simulink model "afe_dqctrl_param"  (R2026a)
settings: Solver=ode23tb  StopTime=param.sim.simlength  FixedStep=tc  MaxStep=param.glb_time.tc
values from neighbouring files (symbols this model uses):
  param = add_template_extras(param, options)    [init_model.m]
undefined symbols (not defined in the file or in its folder): magnitude
libraries: fl_lib x166, nesl_utility x91, igbt_simple_2th_lib x6, single_phase_transformer_lib x3, discrete_time_low_pass_filter x1, threephase_inductor_lib x1, dclink_for_two_levels x1, three_phase_pwm_modulator x1, three_phase_voltage_with_frt_emulator x1
(part 3 of 7)

== system afe_dqctrl_param/afe_dq_mod1/AFE_control/afe_control/acquisitions/ug afe quantizzation and one step delay ==
  ug_abc_pu : Inport
  Demux : Demux  Outputs=3
  Mux : Mux  Inputs=3
  ug afe quantizzation and one step delay : Subsystem
  ugd_abc_pu : Outport
  wires:
  ug afe quantizzation and one step delay/2(ugd_v_pu) -> Mux/2
  Demux/2 -> ug afe quantizzation and one step delay/2(ug_v_pu)
  Demux/3 -> ug afe quantizzation and one step delay/3(ug_w_pu)
  ug afe quantizzation and one step delay/1(ugd_u_pu) -> Mux/1
  Demux/1 -> ug afe quantizzation and one step delay/1(ug_u_pu)
  ug_abc_pu/1 -> Demux/1
  ug afe quantizzation and one step delay/3(ugd_w_pu) -> Mux/3
  Mux/1 -> ugd_abc_pu/1

== system afe_dqctrl_param/afe_dq_mod1/AFE_control/afe_control/current_ctrl/current_transformation ==
  is_a_pu : Inport
  is_b_pu : Inport  Port=2
  is_c_pu : Inport  Port=3
  alphabeta2xieta : MATLAB Function  TreatAsAtomicUnit=on
  uvw2alphabeta : MATLAB Function  TreatAsAtomicUnit=on
  tag scope: id_eta_pu=scoped, id_xi_pu=scoped
  wires:
  is_c_pu/1 -> uvw2alphabeta/3(w)
  alphabeta2xieta/2(eta) -> [id_eta_pu]  "ieta_pu"
  alphabeta2xieta/1(xi) -> [id_xi_pu]  "ixi_pu"
  is_b_pu/1 -> uvw2alphabeta/2(v)
  uvw2alphabeta/2(beta) -> alphabeta2xieta/2(beta)  "ibeta_pu"
  uvw2alphabeta/1(alpha) -> alphabeta2xieta/1(alpha)  "ialpha_pu"
  [phase_grid_pll] -> alphabeta2xieta/3(gamma)
  is_a_pu/1 -> uvw2alphabeta/1(u)

== system afe_dqctrl_param/afe_dq_mod1/AFE_control/afe_control/current_ctrl/dq_vector_pi ==
  id : Inport
  id_ref : Inport  Port=2
  iq : Inport  Port=3
  iq_ref : Inport  Port=4
  Sum1 : Sum  Inputs=|-+
  Sum2 : Sum  Inputs=|-+
  bounder1 : Subsystem
  bounder2 : Subsystem
  pi_d : Subsystem
  pi_q : Subsystem
  switch : Subsystem
  vector lenght : Subsystem
  md_sat : Outport
  mq_sat : Outport  Port=2
  wires:
  bounder2/2(clip) -> switch/2(clip 2)
  vector lenght/2(m) -> bounder1/3(m), bounder2/1(m)
  Sum2/1 -> pi_q/1(iq_tilde)
  pi_d/1(ud_out) -> vector lenght/1(md), bounder1/1(md)
  pi_q/1(Vqs_out) -> bounder2/3(mq), vector lenght/2(mq)
  vector lenght/1(m_1) -> bounder1/2(m_1), bounder2/2(m_1)
  switch/1(clip) -> pi_q/2(clip), pi_d/2(clip)
  iq/1 -> Sum2/1
  Sum1/1 -> pi_d/1(id_tilde)
  bounder1/2(clip) -> switch/1(clip 1)
  id/1 -> Sum1/1
  bounder1/1(md_sat) -> md_sat/1
  bounder2/1(mq_sat) -> mq_sat/1
  id_ref/1 -> Sum1/2
  iq_ref/1 -> Sum2/2

== system afe_dqctrl_param/afe_dq_mod1/AFE_control/afe_control/current_ctrl/zero_current_ctrl ==
  ualpha_ctrl_afe : Inport
  ubeta_ctrl_afe : Inport  Port=2
  Bus Creator1 : BusCreator  Inputs=3
  iz : Subsystem
  zero_sequence_current_ctrl : Subsystem
  uabg_ctrl_out : Outport
  wires:
  Bus Creator1/1 -> uabg_ctrl_out/1
  ualpha_ctrl_afe/1 -> Bus Creator1/1  "ualpha_ctrl_afe"
  ubeta_ctrl_afe/1 -> Bus Creator1/2  "ubeta_ctrl_afe"
  iz/1(iz) -> zero_sequence_current_ctrl/1(iz)
  zero_sequence_current_ctrl/1(ugamma_afe) -> Bus Creator1/3  "ugamma_ctrl_afe"

== system afe_dqctrl_param/afe_dq_mod1/AFE_control/afe_control/data_to_worspace_module_1/dq_pll ==
  Bus Creator1 : BusCreator  Inputs=8
  dqPLLs : Outport
  wires:
  [phase_grid_fht_simulink_pll] -> Bus Creator1/5  "phase_grid_fht_simulink_pll"
  [omega_grid_fht_simulink_pll] -> Bus Creator1/6  "omega_grid_fht_simulink_pll"
  [omega_grid_fhtsr_dqpll] -> Bus Creator1/8  "omega_grid_fhtsr_dqpll"
  [phase_grid_fhtsr_dqpll] -> Bus Creator1/7  "phase_grid_fhtsr_dqpll"
  [omega_grid_dqpll_ccaller] -> Bus Creator1/4  "omega_grid_dqpll_ccaller"
  [phase_grid_dqpll_ccaller] -> Bus Creator1/3  "phase_grid_dqpll_ccaller"
  [omega_grid_pu_dqpll] -> Bus Creator1/2  "omega_grid_pu_dqpll"
  [phase_grid_dqpll] -> Bus Creator1/1  "phase_grid_dqpll"
  Bus Creator1/1 -> dqPLLs/1

== system afe_dqctrl_param/afe_dq_mod1/AFE_control/afe_control/data_to_worspace_module_1/pwr_meter ==
  Bus Creator1 : BusCreator  Inputs=4
  m_pwr_meter : Outport
  wires:
  [u_grid_pu_rms] -> Bus Creator1/2  "u_grid_pu_rms"
  Bus Creator1/1 -> m_pwr_meter/1
  [pwr_act_grid] -> Bus Creator1/3  "pwr_act_grid"
  [pwr_react_grid] -> Bus Creator1/4  "pwr_react_grid"
  [i_grid_pu_rms] -> Bus Creator1/1  "i_grid_pu_rms"

== system afe_dqctrl_param/afe_dq_mod1/AFE_control/afe_control/grid_voltage_phase_lock_loops/FHT-PLL ==
  ug_abc_pu : Inport
  pll_stageA : Subsystem
  pll_stageB : Subsystem
  gamma_grid_fht_pll : Outport
  omega_grid_fht_pll : Outport  Port=2
  wires:
  ug_abc_pu/1 -> pll_stageA/2(ug_abc_pu)
  pll_stageB/2(omega_grid_ddsrf_pll) -> omega_grid_fht_pll/1
  pll_stageA/1(u_grid_xi) -> pll_stageB/1(u_grid_pos_xi)  "u_grid_pos_xi"
  pll_stageA/2(u_grid_eta) -> pll_stageB/2(u_grid_pos_eta)  "u_grid_pos_eta"
  pll_stageB/1(gamma_grid_ddsrf_pll) -> gamma_grid_fht_pll/1, pll_stageA/1(gamma_grid)

== system afe_dqctrl_param/afe_dq_mod1/AFE_control/afe_control/grid_voltage_phase_lock_loops/FHT-PLL_simulink ==
  ug_abc_pu : Inport
  pll_stageA : Subsystem
  pll_stageB : Subsystem
  gamma_grid_fht_pll : Outport
  omega_grid_fht_pll : Outport  Port=2
  wires:
  pll_stageB/1(gamma_grid_ddsrf_pll) -> pll_stageA/1(gamma_grid), gamma_grid_fht_pll/1
  pll_stageA/2(u_grid_eta) -> pll_stageB/2(u_grid_pos_eta)  "u_grid_pos_eta"
  pll_stageA/1(u_grid_xi) -> pll_stageB/1(u_grid_pos_xi)  "u_grid_pos_xi"
  pll_stageB/2(omega_grid_ddsrf_pll) -> omega_grid_fht_pll/1
  ug_abc_pu/1 -> pll_stageA/2(ug_abc_pu)

== system afe_dqctrl_param/afe_dq_mod1/AFE_control/afe_control/grid_voltage_phase_lock_loops/dq_pll ==
  ug_abc_pu : Inport
  Goto Tag Visibility29 : GotoTagVisibility  GotoTag=Vgrid_unorm_dqpll
  pll_stageA : Subsystem
  pll_stageB : Subsystem
  phase_grid_dqpll : Outport
  omega_grid_pu_dqpll : Outport  Port=2
  wires:
  pll_stageA/2(u_grid_pos_eta) -> pll_stageB/2(u_grid_pos_eta)  "u_grid_pos_eta"
  pll_stageB/1(phase_grid_pll) -> phase_grid_dqpll/1, pll_stageA/1(phase_grid)
  pll_stageA/1(u_grid_pos_xi) -> pll_stageB/1(u_grid_pos_xi)  "u_grid_pos_xi"
  pll_stageB/2(omega_grid_pu_pll) -> omega_grid_pu_dqpll/1
  ug_abc_pu/1 -> pll_stageA/2(ug_abc)

== system afe_dqctrl_param/afe_dq_mod1/AFE_control/afe_control/grid_voltage_phase_lock_loops/dq_pll_ccaller ==
  ug_abc_pu : Inport
  Bus Selector : BusSelector  OutputSignals=omega_pu_hat,gamma_hat,u_grid_xi,u_grid_eta,dqpll_pll_state
  C Caller : CCaller  FunctionName=dqpll_grid_process_simulink  PortSpecificationStruct="%)30     .    N H   8    (     @         %    \"     8    !     0         %  0 \"0    $    _    07)G3F%M90  4&]R=$YA;64 4V-O<&4     26YD97@     5'EP90      4VEZ90      27-';&]B86P   X    P    !@    @    $          4    (     0    ,    !         !   P!O=70 #@   #     &    \"     0         !0    @    !     P    $         $  # &]U=  .    .     8    (    !          %    \"     $    &     0         0   ...(+3319 chars)"
  Constant : Constant  Value=param.glb_time.ts_afe
  Data Type Conversion{1..2,4..5} (4 alike) : DataTypeConversion  OutDataTypeStr=single  SaturateOnIntegerOverflow=off  RndMeth=Floor
  Data Type Conversion{6..10} (5 alike) : DataTypeConversion  OutDataTypeStr=double  SaturateOnIntegerOverflow=off  RndMeth=Floor
  Data Type Conversion3 : DataTypeConversion  OutDataTypeStr=uint8  SaturateOnIntegerOverflow=off  RndMeth=Floor
  Demux : Demux  Outputs=3
  Step : Step  Time=0.01  InitialValue=1  FinalValue=0
  first_harmonic_tracker : Scope  NumInputPorts=3
      settings: ActiveDisplayYMinimum=-1.7184470891952515  ActiveDisplayYMaximum=1.8384636640548706
  first_harmonic_tracker_phase_u : Subsystem
  first_harmonic_tracker_phase_v : Subsystem
  first_harmonic_tracker_phase_w : Subsystem
  gamma_hat : Outport  VectorParamsAs1DForOutWhenUnconnected=off
  omega_pu_hat : Outport  Port=2  VectorParamsAs1DForOutWhenUnconnected=off
  dqpll_uxi : Outport  Port=3  VectorParamsAs1DForOutWhenUnconnected=off
  dqpll_ueta : Outport  Port=4  VectorParamsAs1DForOutWhenUnconnected=off
  dqpll_state : Outport  Port=5  VectorParamsAs1DForOutWhenUnconnected=off
  wires:
  Step/1 -> Data Type Conversion3/1
  Constant/1 -> Data Type Conversion1/1
  Data Type Conversion3/1 -> C Caller/1
  Data Type Conversion2/1 -> C Caller/2
  Data Type Conversion4/1 -> C Caller/3
  Data Type Conversion5/1 -> C Caller/4
  Data Type Conversion1/1 -> C Caller/5
  C Caller/1 -> Bus Selector/1
  Bus Selector/1 -> Data Type Conversion6/1  "<omega_pu_hat>"
  Bus Selector/2 -> Data Type Conversion7/1  "<gamma_hat>"
  Bus Selector/3 -> Data Type Conversion8/1  "<u_grid_xi>"
  Bus Selector/4 -> Data Type Conversion9/1  "<u_grid_eta>"
  Bus Selector/5 -> Data Type Conversion10/1  "<dqpll_pll_state>"
  Data Type Conversion7/1 -> gamma_hat/1
  Data Type Conversion10/1 -> dqpll_state/1
  Data Type Conversion8/1 -> dqpll_uxi/1
  Data Type Conversion9/1 -> dqpll_ueta/1
  ug_abc_pu/1 -> Demux/1
  Demux/1 -> first_harmonic_tracker_phase_u/1(u)
  Demux/2 -> first_harmonic_tracker_phase_v/1(u)
  Demux/3 -> first_harmonic_tracker_phase_w/1(u)
  Data Type Conversion6/1 -> omega_pu_hat/1
  first_harmonic_tracker_phase_u/1(u_hat) -> first_harmonic_tracker/1, Data Type Conversion2/1  "tracker_phase_u"
  first_harmonic_tracker_phase_v/1(u_hat) -> first_harmonic_tracker/2, Data Type Conversion4/1  "tracker_phase_v"
  first_harmonic_tracker_phase_w/1(u_hat) -> first_harmonic_tracker/3, Data Type Conversion5/1  "tracker_phase_w"

== system afe_dqctrl_param/afe_dq_mod1/AFE_control/afe_control/instantaneus_power/abc2alphabeta ==
  a : Inport
  b : Inport  Port=2
  c : Inport  Port=3
  Gain1 : Gain  Gain=-1/2
  Gain11 : Gain  Gain=-1/2
  Gain2 : Gain  Gain=0
  Gain3 : Gain  Gain=sqrt(3)/2
  Gain4 : Gain  Gain=-sqrt(3)/2
  Gain8 : Gain  Gain=2/3
  Gain9 : Gain  Gain=2/3
  Sum : Sum  Inputs=+++
  Sum1 : Sum  Inputs=+++
  "alpha " : Outport  VectorParamsAs1DForOutWhenUnconnected=off
  "beta " : Outport  Port=2  VectorParamsAs1DForOutWhenUnconnected=off
  wires:
  Gain3/1 -> Sum1/2
  Gain2/1 -> Sum1/1
  Gain11/1 -> Sum/2
  Gain4/1 -> Sum1/3
  Sum1/1 -> Gain9/1
  Gain8/1 -> "alpha "/1
  Sum/1 -> Gain8/1
  c/1 -> Gain4/1, Gain1/1
  Gain9/1 -> "beta "/1
  b/1 -> Gain3/1, Gain11/1
  Gain1/1 -> Sum/3
  a/1 -> Gain2/1, Sum/1

== system afe_dqctrl_param/afe_dq_mod1/AFE_control/afe_control/instantaneus_power/abc2alphabeta  ==
  a : Inport
  b : Inport  Port=2
  c : Inport  Port=3
  Gain1 : Gain  Gain=-1/2
  Gain11 : Gain  Gain=-1/2
  Gain2 : Gain  Gain=0
  Gain3 : Gain  Gain=sqrt(3)/2
  Gain4 : Gain  Gain=-sqrt(3)/2
  Gain8 : Gain  Gain=2/3
  Gain9 : Gain  Gain=2/3
  Sum : Sum  Inputs=+++
  Sum1 : Sum  Inputs=+++
  "alpha " : Outport  VectorParamsAs1DForOutWhenUnconnected=off
  "beta " : Outport  Port=2  VectorParamsAs1DForOutWhenUnconnected=off
  wires:
  a/1 -> Sum/1, Gain2/1
  Gain2/1 -> Sum1/1
  Gain9/1 -> "beta "/1
  Gain11/1 -> Sum/2
  c/1 -> Gain1/1, Gain4/1
  Sum/1 -> Gain8/1
  Sum1/1 -> Gain9/1
  Gain1/1 -> Sum/3
  Gain3/1 -> Sum1/2
  Gain4/1 -> Sum1/3
  Gain8/1 -> "alpha "/1
  b/1 -> Gain11/1, Gain3/1

== system afe_dqctrl_param/afe_dq_mod1/AFE_control/afe_control/instantaneus_power/moving_avarage_p ==
  in : Inport
  Gain : Gain  Gain=param.afe.ctrl.rms.n1-1
  Gain1 : Gain  Gain=1/param.afe.ctrl.rms.n1
  Sum : Sum  Inputs=|++
  Unit Delay : UnitDelay  SampleTime=-1
  out : Outport  VectorParamsAs1DForOutWhenUnconnected=off
  wires:
  Gain/1 -> Sum/2
  Gain1/1 -> out/1, Unit Delay/1
  in/1 -> Sum/1
  Unit Delay/1 -> Gain/1
  Sum/1 -> Gain1/1

== system afe_dqctrl_param/afe_dq_mod1/AFE_control/afe_control/instantaneus_power/moving_avarage_q ==
  in : Inport
  Gain : Gain  Gain=param.afe.ctrl.rms.n1-1
  Gain1 : Gain  Gain=1/param.afe.ctrl.rms.n1
  Sum : Sum  Inputs=|++
  Unit Delay : UnitDelay  SampleTime=-1
  out : Outport  VectorParamsAs1DForOutWhenUnconnected=off
  wires:
  Sum/1 -> Gain1/1
  Unit Delay/1 -> Gain/1
  in/1 -> Sum/1
  Gain1/1 -> Unit Delay/1, out/1
  Gain/1 -> Sum/2

== system afe_dqctrl_param/afe_dq_mod1/AFE_control/afe_control/instantaneus_power/rms ==
  In1 : Inport
  Gain : Gain  Gain=param.afe.ctrl.rms.n10-1
  Gain1 : Gain  Gain=1/param.afe.ctrl.rms.n10
  Math Function : Math  Operator=magnitude^2  SignedPower=on
  Sqrt : Sqrt
  Sum : Sum  Inputs=|++
  Unit Delay : UnitDelay  SampleTime=-1
  Out1 : Outport  VectorParamsAs1DForOutWhenUnconnected=off
  wires:
  In1/1 -> Math Function/1
  Sum/1 -> Gain1/1
  Gain1/1 -> Sqrt/1, Unit Delay/1
  Unit Delay/1 -> Gain/1
  Math Function/1 -> Sum/1
  Sqrt/1 -> Out1/1
  Gain/1 -> Sum/2

== system afe_dqctrl_param/afe_dq_mod1/AFE_control/afe_control/instantaneus_power/rms1 ==
  In1 : Inport
  Gain : Gain  Gain=param.afe.ctrl.rms.n10-1
  Gain1 : Gain  Gain=1/param.afe.ctrl.rms.n10
  Math Function : Math  Operator=magnitude^2  SignedPower=on
  Sqrt : Sqrt
  Sum : Sum  Inputs=|++
  Unit Delay : UnitDelay  SampleTime=-1
  Out1 : Outport  VectorParamsAs1DForOutWhenUnconnected=off
  wires:
  Gain/1 -> Sum/2
  Sqrt/1 -> Out1/1
  Math Function/1 -> Sum/1
  Unit Delay/1 -> Gain/1
  Gain1/1 -> Unit Delay/1, Sqrt/1
  Sum/1 -> Gain1/1
  In1/1 -> Math Function/1

== system afe_dqctrl_param/afe_dq_mod1/AFE_control/afe_control/instantaneus_power/rms2 ==
  In1 : Inport
  Gain : Gain  Gain=param.afe.ctrl.rms.n10-1
  Gain1 : Gain  Gain=1/param.afe.ctrl.rms.n10
  Math Function : Math  Operator=magnitude^2  SignedPower=on
  Sqrt : Sqrt
  Sum : Sum  Inputs=|++
  Unit Delay : UnitDelay  SampleTime=-1
  Out1 : Outport  VectorParamsAs1DForOutWhenUnconnected=off
  wires:
  In1/1 -> Math Function/1
  Sum/1 -> Gain1/1
  Gain1/1 -> Sqrt/1, Unit Delay/1
  Unit Delay/1 -> Gain/1
  Math Function/1 -> Sum/1
  Sqrt/1 -> Out1/1
  Gain/1 -> Sum/2

== system afe_dqctrl_param/afe_dq_mod1/AFE_control/afe_control/instantaneus_power/rms3 ==
  In1 : Inport
  Gain : Gain  Gain=param.afe.ctrl.rms.n10-1
  Gain1 : Gain  Gain=1/param.afe.ctrl.rms.n10
  Math Function : Math  Operator=magnitude^2  SignedPower=on
  Sqrt : Sqrt
  Sum : Sum  Inputs=|++
  Unit Delay : UnitDelay  SampleTime=-1
  Out1 : Outport  VectorParamsAs1DForOutWhenUnconnected=off
  wires:
  Gain/1 -> Sum/2
  Sqrt/1 -> Out1/1
  Math Function/1 -> Sum/1
  Unit Delay/1 -> Gain/1
  Gain1/1 -> Unit Delay/1, Sqrt/1
  Sum/1 -> Gain1/1
  In1/1 -> Math Function/1

== system afe_dqctrl_param/afe_dq_mod1/AFE_control/afe_control/instantaneus_power/rms4 ==
  In1 : Inport
  Gain : Gain  Gain=param.afe.ctrl.rms.n10-1
  Gain1 : Gain  Gain=1/param.afe.ctrl.rms.n10
  Math Function : Math  Operator=magnitude^2  SignedPower=on
  Sqrt : Sqrt
  Sum : Sum  Inputs=|++
  Unit Delay : UnitDelay  SampleTime=-1
  Out1 : Outport  VectorParamsAs1DForOutWhenUnconnected=off
  wires:
  In1/1 -> Math Function/1
  Sum/1 -> Gain1/1
  Gain1/1 -> Sqrt/1, Unit Delay/1
  Unit Delay/1 -> Gain/1
  Math Function/1 -> Sum/1
  Sqrt/1 -> Out1/1
  Gain/1 -> Sum/2

== system afe_dqctrl_param/afe_dq_mod1/AFE_control/afe_control/instantaneus_power/rms5 ==
  In1 : Inport
  Gain : Gain  Gain=param.afe.ctrl.rms.n10-1
  Gain1 : Gain  Gain=1/param.afe.ctrl.rms.n10
  Math Function : Math  Operator=magnitude^2  SignedPower=on
  Sqrt : Sqrt
  Sum : Sum  Inputs=|++
  Unit Delay : UnitDelay  SampleTime=-1
  Out1 : Outport  VectorParamsAs1DForOutWhenUnconnected=off
  wires:
  Gain/1 -> Sum/2
  Sqrt/1 -> Out1/1
  Math Function/1 -> Sum/1
  Unit Delay/1 -> Gain/1
  Gain1/1 -> Unit Delay/1, Sqrt/1
  Sum/1 -> Gain1/1
  In1/1 -> Math Function/1

== system afe_dqctrl_param/afe_dq_mod1/afe/three_phase_inverter_with_igbt_simple_2th/three_phase_inverter_with_igbt_simple_2th/igbt_simple_1 ==
  note: P_sw
  Capacitor : fl_lib/Electrical/Electrical Elements/Capacitor  c=Csnubber_m F  r=Rsnubber_m Ohm  g=0 1/Ohm  i_specify=off  i_priority=None  i=0 A  i_nominal_specify=off  i_nominal_value=1  i_nominal_unit=A  v_specify=off  v_priority=None  v=0 V  v_nominal_specify=off  v_nominal_value=1  v_nominal_unit=V  vc_specify=off  vc_priority=High  vc=0 V  vc_nominal_specify=off  vc_nominal_value=1  vc_nominal_unit=V
  IGBT_simple : Subsystem
      settings: PortSchema="{\"entries\":[{\"content\":{\"sides\":[{\"content\":{\"connectorIds\":[\"LConn1\"]},\"type\":\"ConnectorPlacement.EquallySpacedRectSide\",\"uuid\":\"c3d88d60-081d-4221-ab18-079856838dba\"},{\"content\":{\"side\":\"RIGHT\"},\"type\":\"ConnectorPlacement.EquallySpacedRectSide\",\"uuid\":\"76e7d76c-8b60-4107-8aac-a7654bd886e1\"},{\"content\":{\"connectorIds\":[\"LConn2\"],\"side\":\"TOP\"},\"type\":\"ConnectorPlacement.EquallySpacedRectSide\",\"uuid\":\"fbef57e1-7143-4076-ada8-0654b1d9ee0b\"},{\"content\":{\"connectorIds\":[\"RConn1\"],\"side\":\"BOTTOM\"},\"type\":\"ConnectorPlacement.EquallySpacedRectSide\",\"uuid\":\"f2fea5db-9515-452a-a480-7d54bae36c49\"}]},\"type\":\"ConnectorPlacement.EquallySpacedConnector\",\"uuid\":\"cddff0b8-236e-4840-ad87-03abcdd65fe7\"}],\"packageUris\":[\"http://schema.mathworks.com/mf0/Connector/R2020b\"],\"version\":\"1.0\"}"
  Voltage Sensor : fl_lib/Electrical/Electrical Sensors/Voltage Sensor
  uph : nesl_utility/PS-Simulink Converter  PhysicalDomain=network_engine_domain  SubClassName=ps_output  LeftPortType=input  RightPortType=output  PseudoPeriodic=off  Frequencies=[]  VectorFormat=1-D array  Unit=V  AffineConversion=off
  G : PMIOPort  Side=Left
  C : PMIOPort  Port=2  Side=Left
  E : PMIOPort  Port=3  Side=Right
  tag scope: igbt_voltage_Q1=scoped
  wires:
  uph/1 -> [igbt_voltage_Q1]  "uph"
  connections:
  G/RConn1 -- IGBT_simple/LConn1
  Voltage Sensor/RConn1 -- uph/LConn1
  Capacitor/LConn1 -- Voltage Sensor/LConn1 -- C/RConn1 -- IGBT_simple/LConn2
  Capacitor/RConn1 -- Voltage Sensor/RConn2 -- E/RConn1 -- IGBT_simple/RConn1

== system afe_dqctrl_param/afe_dq_mod1/afe/three_phase_inverter_with_igbt_simple_2th/three_phase_inverter_with_igbt_simple_2th/igbt_simple_2 ==
  note: P_sw
  Capacitor : fl_lib/Electrical/Electrical Elements/Capacitor  c=Csnubber_m F  r=Rsnubber_m Ohm  g=0 1/Ohm  i_specify=off  i_priority=None  i=0 A  i_nominal_specify=off  i_nominal_value=1  i_nominal_unit=A  v_specify=off  v_priority=None  v=0 V  v_nominal_specify=off  v_nominal_value=1  v_nominal_unit=V  vc_specify=off  vc_priority=High  vc=0 V  vc_nominal_specify=off  vc_nominal_value=1  vc_nominal_unit=V
  IGBT_simple : Subsystem
      settings: PortSchema="{\"entries\":[{\"content\":{\"sides\":[{\"content\":{\"connectorIds\":[\"LConn1\"]},\"type\":\"ConnectorPlacement.EquallySpacedRectSide\",\"uuid\":\"c3d88d60-081d-4221-ab18-079856838dba\"},{\"content\":{\"side\":\"RIGHT\"},\"type\":\"ConnectorPlacement.EquallySpacedRectSide\",\"uuid\":\"76e7d76c-8b60-4107-8aac-a7654bd886e1\"},{\"content\":{\"connectorIds\":[\"LConn2\"],\"side\":\"TOP\"},\"type\":\"ConnectorPlacement.EquallySpacedRectSide\",\"uuid\":\"fbef57e1-7143-4076-ada8-0654b1d9ee0b\"},{\"content\":{\"connectorIds\":[\"RConn1\"],\"side\":\"BOTTOM\"},\"type\":\"ConnectorPlacement.EquallySpacedRectSide\",\"uuid\":\"f2fea5db-9515-452a-a480-7d54bae36c49\"}]},\"type\":\"ConnectorPlacement.EquallySpacedConnector\",\"uuid\":\"cddff0b8-236e-4840-ad87-03abcdd65fe7\"}],\"packageUris\":[\"http://schema.mathworks.com/mf0/Connector/R2020b\"],\"version\":\"1.0\"}"
  Voltage Sensor : fl_lib/Electrical/Electrical Sensors/Voltage Sensor
  uph : nesl_utility/PS-Simulink Converter  PhysicalDomain=network_engine_domain  SubClassName=ps_output  LeftPortType=input  RightPortType=output  PseudoPeriodic=off  Frequencies=[]  VectorFormat=1-D array  Unit=V  AffineConversion=off
  G : PMIOPort  Side=Left
  C : PMIOPort  Port=2  Side=Left
  E : PMIOPort  Port=3  Side=Right
  tag scope: igbt_voltage_Q2=scoped
  wires:
  uph/1 -> [igbt_voltage_Q2]  "uph"
  connections:
  IGBT_simple/RConn1 -- E/RConn1 -- Capacitor/RConn1 -- Voltage Sensor/RConn2
  C/RConn1 -- IGBT_simple/LConn2 -- Capacitor/LConn1 -- Voltage Sensor/LConn1
  Voltage Sensor/RConn1 -- uph/LConn1
  G/RConn1 -- IGBT_simple/LConn1

== system afe_dqctrl_param/afe_dq_mod1/afe/three_phase_inverter_with_igbt_simple_2th/three_phase_inverter_with_igbt_simple_2th/igbt_simple_3 ==
  note: P_sw
  Capacitor : fl_lib/Electrical/Electrical Elements/Capacitor  c=Csnubber_m F  r=Rsnubber_m Ohm  g=0 1/Ohm  i_specify=off  i_priority=None  i=0 A  i_nominal_specify=off  i_nominal_value=1  i_nominal_unit=A  v_specify=off  v_priority=None  v=0 V  v_nominal_specify=off  v_nominal_value=1  v_nominal_unit=V  vc_specify=off  vc_priority=High  vc=0 V  vc_nominal_specify=off  vc_nominal_value=1  vc_nominal_unit=V
  IGBT_simple : Subsystem
      settings: PortSchema="{\"entries\":[{\"content\":{\"sides\":[{\"content\":{\"connectorIds\":[\"LConn1\"]},\"type\":\"ConnectorPlacement.EquallySpacedRectSide\",\"uuid\":\"c3d88d60-081d-4221-ab18-079856838dba\"},{\"content\":{\"side\":\"RIGHT\"},\"type\":\"ConnectorPlacement.EquallySpacedRectSide\",\"uuid\":\"76e7d76c-8b60-4107-8aac-a7654bd886e1\"},{\"content\":{\"connectorIds\":[\"LConn2\"],\"side\":\"TOP\"},\"type\":\"ConnectorPlacement.EquallySpacedRectSide\",\"uuid\":\"fbef57e1-7143-4076-ada8-0654b1d9ee0b\"},{\"content\":{\"connectorIds\":[\"RConn1\"],\"side\":\"BOTTOM\"},\"type\":\"ConnectorPlacement.EquallySpacedRectSide\",\"uuid\":\"f2fea5db-9515-452a-a480-7d54bae36c49\"}]},\"type\":\"ConnectorPlacement.EquallySpacedConnector\",\"uuid\":\"cddff0b8-236e-4840-ad87-03abcdd65fe7\"}],\"packageUris\":[\"http://schema.mathworks.com/mf0/Connector/R2020b\"],\"version\":\"1.0\"}"
  Voltage Sensor : fl_lib/Electrical/Electrical Sensors/Voltage Sensor
  uph : nesl_utility/PS-Simulink Converter  PhysicalDomain=network_engine_domain  SubClassName=ps_output  LeftPortType=input  RightPortType=output  PseudoPeriodic=off  Frequencies=[]  VectorFormat=1-D array  Unit=V  AffineConversion=off
  G : PMIOPort  Side=Left
  C : PMIOPort  Port=2  Side=Left
  E : PMIOPort  Port=3  Side=Right
  tag scope: igbt_voltage_Q3=scoped
  wires:
  uph/1 -> [igbt_voltage_Q3]  "uph"
  connections:
  G/RConn1 -- IGBT_simple/LConn1
  Voltage Sensor/RConn1 -- uph/LConn1
  Voltage Sensor/LConn1 -- Capacitor/LConn1 -- IGBT_simple/LConn2 -- C/RConn1
  Voltage Sensor/RConn2 -- Capacitor/RConn1 -- E/RConn1 -- IGBT_simple/RConn1

== system afe_dqctrl_param/afe_dq_mod1/afe/three_phase_inverter_with_igbt_simple_2th/three_phase_inverter_with_igbt_simple_2th/igbt_simple_4 ==
  note: P_sw
  Capacitor : fl_lib/Electrical/Electrical Elements/Capacitor  c=Csnubber_m F  r=Rsnubber_m Ohm  g=0 1/Ohm  i_specify=off  i_priority=None  i=0 A  i_nominal_specify=off  i_nominal_value=1  i_nominal_unit=A  v_specify=off  v_priority=None  v=0 V  v_nominal_specify=off  v_nominal_value=1  v_nominal_unit=V  vc_specify=off  vc_priority=High  vc=0 V  vc_nominal_specify=off  vc_nominal_value=1  vc_nominal_unit=V
  IGBT_simple : Subsystem
      settings: PortSchema="{\"entries\":[{\"content\":{\"sides\":[{\"content\":{\"connectorIds\":[\"LConn1\"]},\"type\":\"ConnectorPlacement.EquallySpacedRectSide\",\"uuid\":\"c3d88d60-081d-4221-ab18-079856838dba\"},{\"content\":{\"side\":\"RIGHT\"},\"type\":\"ConnectorPlacement.EquallySpacedRectSide\",\"uuid\":\"76e7d76c-8b60-4107-8aac-a7654bd886e1\"},{\"content\":{\"connectorIds\":[\"LConn2\"],\"side\":\"TOP\"},\"type\":\"ConnectorPlacement.EquallySpacedRectSide\",\"uuid\":\"fbef57e1-7143-4076-ada8-0654b1d9ee0b\"},{\"content\":{\"connectorIds\":[\"RConn1\"],\"side\":\"BOTTOM\"},\"type\":\"ConnectorPlacement.EquallySpacedRectSide\",\"uuid\":\"f2fea5db-9515-452a-a480-7d54bae36c49\"}]},\"type\":\"ConnectorPlacement.EquallySpacedConnector\",\"uuid\":\"cddff0b8-236e-4840-ad87-03abcdd65fe7\"}],\"packageUris\":[\"http://schema.mathworks.com/mf0/Connector/R2020b\"],\"version\":\"1.0\"}"
  Voltage Sensor : fl_lib/Electrical/Electrical Sensors/Voltage Sensor
  uph : nesl_utility/PS-Simulink Converter  PhysicalDomain=network_engine_domain  SubClassName=ps_output  LeftPortType=input  RightPortType=output  PseudoPeriodic=off  Frequencies=[]  VectorFormat=1-D array  Unit=V  AffineConversion=off
  G : PMIOPort  Side=Left
  C : PMIOPort  Port=2  Side=Left
  E : PMIOPort  Port=3  Side=Right
  tag scope: igbt_voltage_Q4=scoped
  wires:
  uph/1 -> [igbt_voltage_Q4]  "uph"
  connections:
  IGBT_simple/RConn1 -- E/RConn1 -- Capacitor/RConn1 -- Voltage Sensor/RConn2
  C/RConn1 -- IGBT_simple/LConn2 -- Capacitor/LConn1 -- Voltage Sensor/LConn1
  Voltage Sensor/RConn1 -- uph/LConn1
  G/RConn1 -- IGBT_simple/LConn1

== system afe_dqctrl_param/afe_dq_mod1/afe/three_phase_inverter_with_igbt_simple_2th/three_phase_inverter_with_igbt_simple_2th/igbt_simple_5 ==
  note: P_sw
  Capacitor : fl_lib/Electrical/Electrical Elements/Capacitor  c=Csnubber_m F  r=Rsnubber_m Ohm  g=0 1/Ohm  i_specify=off  i_priority=None  i=0 A  i_nominal_specify=off  i_nominal_value=1  i_nominal_unit=A  v_specify=off  v_priority=None  v=0 V  v_nominal_specify=off  v_nominal_value=1  v_nominal_unit=V  vc_specify=off  vc_priority=High  vc=0 V  vc_nominal_specify=off  vc_nominal_value=1  vc_nominal_unit=V
  IGBT_simple : Subsystem
      settings: PortSchema="{\"entries\":[{\"content\":{\"sides\":[{\"content\":{\"connectorIds\":[\"LConn1\"]},\"type\":\"ConnectorPlacement.EquallySpacedRectSide\",\"uuid\":\"c3d88d60-081d-4221-ab18-079856838dba\"},{\"content\":{\"side\":\"RIGHT\"},\"type\":\"ConnectorPlacement.EquallySpacedRectSide\",\"uuid\":\"76e7d76c-8b60-4107-8aac-a7654bd886e1\"},{\"content\":{\"connectorIds\":[\"LConn2\"],\"side\":\"TOP\"},\"type\":\"ConnectorPlacement.EquallySpacedRectSide\",\"uuid\":\"fbef57e1-7143-4076-ada8-0654b1d9ee0b\"},{\"content\":{\"connectorIds\":[\"RConn1\"],\"side\":\"BOTTOM\"},\"type\":\"ConnectorPlacement.EquallySpacedRectSide\",\"uuid\":\"f2fea5db-9515-452a-a480-7d54bae36c49\"}]},\"type\":\"ConnectorPlacement.EquallySpacedConnector\",\"uuid\":\"cddff0b8-236e-4840-ad87-03abcdd65fe7\"}],\"packageUris\":[\"http://schema.mathworks.com/mf0/Connector/R2020b\"],\"version\":\"1.0\"}"
  Voltage Sensor : fl_lib/Electrical/Electrical Sensors/Voltage Sensor
  uph : nesl_utility/PS-Simulink Converter  PhysicalDomain=network_engine_domain  SubClassName=ps_output  LeftPortType=input  RightPortType=output  PseudoPeriodic=off  Frequencies=[]  VectorFormat=1-D array  Unit=V  AffineConversion=off
  G : PMIOPort  Side=Left
  C : PMIOPort  Port=2  Side=Left
  E : PMIOPort  Port=3  Side=Right
  tag scope: igbt_voltage_Q5=scoped
  wires:
  uph/1 -> [igbt_voltage_Q5]  "uph"
  connections:
  G/RConn1 -- IGBT_simple/LConn1
  Voltage Sensor/RConn1 -- uph/LConn1
  Voltage Sensor/LConn1 -- Capacitor/LConn1 -- IGBT_simple/LConn2 -- C/RConn1
  Voltage Sensor/RConn2 -- Capacitor/RConn1 -- E/RConn1 -- IGBT_simple/RConn1

== system afe_dqctrl_param/afe_dq_mod1/afe/three_phase_inverter_with_igbt_simple_2th/three_phase_inverter_with_igbt_simple_2th/igbt_simple_6 ==
  note: P_sw
  Capacitor : fl_lib/Electrical/Electrical Elements/Capacitor  c=Csnubber_m F  r=Rsnubber_m Ohm  g=0 1/Ohm  i_specify=off  i_priority=None  i=0 A  i_nominal_specify=off  i_nominal_value=1  i_nominal_unit=A  v_specify=off  v_priority=None  v=0 V  v_nominal_specify=off  v_nominal_value=1  v_nominal_unit=V  vc_specify=off  vc_priority=High  vc=0 V  vc_nominal_specify=off  vc_nominal_value=1  vc_nominal_unit=V
  IGBT_simple : Subsystem
      settings: PortSchema="{\"entries\":[{\"content\":{\"sides\":[{\"content\":{\"connectorIds\":[\"LConn1\"]},\"type\":\"ConnectorPlacement.EquallySpacedRectSide\",\"uuid\":\"c3d88d60-081d-4221-ab18-079856838dba\"},{\"content\":{\"side\":\"RIGHT\"},\"type\":\"ConnectorPlacement.EquallySpacedRectSide\",\"uuid\":\"76e7d76c-8b60-4107-8aac-a7654bd886e1\"},{\"content\":{\"connectorIds\":[\"LConn2\"],\"side\":\"TOP\"},\"type\":\"ConnectorPlacement.EquallySpacedRectSide\",\"uuid\":\"fbef57e1-7143-4076-ada8-0654b1d9ee0b\"},{\"content\":{\"connectorIds\":[\"RConn1\"],\"side\":\"BOTTOM\"},\"type\":\"ConnectorPlacement.EquallySpacedRectSide\",\"uuid\":\"f2fea5db-9515-452a-a480-7d54bae36c49\"}]},\"type\":\"ConnectorPlacement.EquallySpacedConnector\",\"uuid\":\"cddff0b8-236e-4840-ad87-03abcdd65fe7\"}],\"packageUris\":[\"http://schema.mathworks.com/mf0/Connector/R2020b\"],\"version\":\"1.0\"}"
  Voltage Sensor : fl_lib/Electrical/Electrical Sensors/Voltage Sensor
  uph : nesl_utility/PS-Simulink Converter  PhysicalDomain=network_engine_domain  SubClassName=ps_output  LeftPortType=input  RightPortType=output  PseudoPeriodic=off  Frequencies=[]  VectorFormat=1-D array  Unit=V  AffineConversion=off
  G : PMIOPort  Side=Left
  C : PMIOPort  Port=2  Side=Left
  E : PMIOPort  Port=3  Side=Right
  tag scope: igbt_voltage_Q6=scoped
  wires:
  uph/1 -> [igbt_voltage_Q6]  "uph"
  connections:
  IGBT_simple/RConn1 -- E/RConn1 -- Capacitor/RConn1 -- Voltage Sensor/RConn2
  C/RConn1 -- IGBT_simple/LConn2 -- Capacitor/LConn1 -- Voltage Sensor/LConn1
  Voltage Sensor/RConn1 -- uph/LConn1
  G/RConn1 -- IGBT_simple/LConn1

== system afe_dqctrl_param/afe_dq_mod1/afe/three_phase_inverter_with_igbt_simple_2th/three_phase_inverter_with_igbt_simple_2th/module_1 ==
  Bus Creator : BusCreator  Inputs=18
  m : Outport
  wires:
  [diode_HA_temp_Q1] -> Bus Creator/8  "diode_HA_temp_Q1"
  [igbt_voltage_Q2] -> Bus Creator/10  "igbt_voltage_Q2"
  [igbt_voltage_Q1] -> Bus Creator/2  "igbt_voltage_Q1"
  [igbt_ploss_Q2] -> Bus Creator/9  "igbt_ploss_Q2"
  [igbt_current_Q2] -> Bus Creator/11  "igbt_current_Q2"
  [diode_ploss_Q1] -> Bus Creator/6  "diode_ploss_Q1"
  [diode_JH_temp_Q1] -> Bus Creator/7  "diode_JH_temp_Q1"
  [igbt_HA_temp_Q1] -> Bus Creator/5  "igbt_HA_temp_Q1"
  [igbt_ploss_Q1] -> Bus Creator/1  "igbt_ploss_Q1"
  [diode_JH_temp_Q2] -> Bus Creator/15  "diode_JH_temp_Q2"
  [diode_HA_temp_Q2] -> Bus Creator/16  "diode_HA_temp_Q2"
  [diode_ploss_Q2] -> Bus Creator/14  "diode_ploss_Q2"
  [igbt_HA_temp_Q2] -> Bus Creator/13  "igbt_HA_temp_Q2"
  [igbt_JH_temp_Q2] -> Bus Creator/12  "igbt_JH_temp_Q2"
  [igbt_JH_temp_Q1] -> Bus Creator/4  "igbt_JH_temp_Q1"
  [igbt_current_Q1] -> Bus Creator/3  "igbt_current_Q1"
  Bus Creator/1 -> m/1  "module_1"
  [diode_current_Q1] -> Bus Creator/17  "diode_current_Q1"
  [diode_current_Q2] -> Bus Creator/18  "diode_current_Q2"

== system afe_dqctrl_param/afe_dq_mod1/afe/three_phase_inverter_with_igbt_simple_2th/three_phase_inverter_with_igbt_simple_2th/module_2 ==
  Bus Creator1 : BusCreator  Inputs=18
  m : Outport
  wires:
  [diode_HA_temp_Q4] -> Bus Creator1/16  "diode_HA_temp_Q4"
  [igbt_HA_temp_Q3] -> Bus Creator1/5  "igbt_HA_temp_Q3"
  [igbt_JH_temp_Q3] -> Bus Creator1/4  "igbt_JH_temp_Q3"
  [diode_ploss_Q3] -> Bus Creator1/6  "diode_ploss_Q3"
  [diode_JH_temp_Q4] -> Bus Creator1/15  "diode_JH_temp_Q4"
  [igbt_ploss_Q3] -> Bus Creator1/1  "igbt_ploss_Q3"
  [igbt_JH_temp_Q4] -> Bus Creator1/12  "igbt_JH_temp_Q4"
  [igbt_voltage_Q3] -> Bus Creator1/2  "igbt_voltage_Q3"
  [igbt_current_Q4] -> Bus Creator1/11  "igbt_current_Q4"
  [diode_HA_temp_Q3] -> Bus Creator1/8  "diode_HA_temp_Q3"
  [igbt_voltage_Q4] -> Bus Creator1/10  "igbt_voltage_Q4"
  [igbt_ploss_Q4] -> Bus Creator1/9  "igbt_ploss_Q4"
  [igbt_HA_temp_Q4] -> Bus Creator1/13  "igbt_HA_temp_Q4"
  [diode_JH_temp_Q3] -> Bus Creator1/7  "diode_JH_temp_Q3"
  [diode_ploss_Q4] -> Bus Creator1/14  "diode_ploss_Q4"
  [igbt_current_Q3] -> Bus Creator1/3  "igbt_current_Q3"
  Bus Creator1/1 -> m/1  "module_2"
  [diode_current_Q4] -> Bus Creator1/18  "diode_current_Q4"
  [diode_current_Q3] -> Bus Creator1/17  "diode_current_Q3"

== system afe_dqctrl_param/afe_dq_mod1/afe/three_phase_inverter_with_igbt_simple_2th/three_phase_inverter_with_igbt_simple_2th/module_3 ==
  Bus Creator1 : BusCreator  Inputs=18
  m : Outport
  wires:
  [diode_ploss_Q6] -> Bus Creator1/14  "diode_ploss_Q6"
  [igbt_HA_temp_Q5] -> Bus Creator1/5  "igbt_HA_temp_Q5"
  [igbt_voltage_Q6] -> Bus Creator1/10  "igbt_voltage_Q6"
  [igbt_voltage_Q5] -> Bus Creator1/2  "igbt_voltage_Q5"
  [igbt_JH_temp_Q6] -> Bus Creator1/12  "igbt_JH_temp_Q6"
  [igbt_current_Q6] -> Bus Creator1/11  "igbt_current_Q6"
  [diode_JH_temp_Q6] -> Bus Creator1/15  "diode_JH_temp_Q6"
  [diode_HA_temp_Q5] -> Bus Creator1/8  "diode_HA_temp_Q5"
  [igbt_ploss_Q5] -> Bus Creator1/1  "igbt_ploss_Q5"
  [igbt_ploss_Q6] -> Bus Creator1/9  "igbt_ploss_Q6"
  [igbt_current_Q5] -> Bus Creator1/3  "igbt_current_Q5"
  [diode_JH_temp_Q5] -> Bus Creator1/7  "diode_JH_temp_Q5"
  [igbt_JH_temp_Q5] -> Bus Creator1/4  "igbt_JH_temp_Q5"
  [diode_HA_temp_Q6] -> Bus Creator1/16  "diode_HA_temp_Q6"
  [igbt_HA_temp_Q6] -> Bus Creator1/13  "igbt_HA_temp_Q6"
  [diode_ploss_Q5] -> Bus Creator1/6  "diode_ploss_Q5"
  Bus Creator1/1 -> m/1  "module_3"
  [diode_current_Q6] -> Bus Creator1/18  "diode_current_Q6"
  [diode_current_Q5] -> Bus Creator1/17  "diode_current_Q5"

== system afe_dqctrl_param/afe_dq_mod1/AFE_control/afe_control/acquisitions/ig afe quantizzation and one step delay/ig afe quantizzation and one step delay ==
  ig_u_pu : Inport
  ig_v_pu : Inport  Port=2
  ig_w_pu : Inport  Port=3
  Gain4 : Gain  Gain=-1
  Gain5 : Gain  Gain=-1
  Gain6 : Gain  Gain=-1
  Quantizer1 : Quantizer  QuantizationInterval=param.meas.adc_quantization
  Quantizer2 : Quantizer  QuantizationInterval=param.meas.adc_quantization
  Quantizer4 : Quantizer  QuantizationInterval=param.meas.adc_quantization
  Unit Delay : UnitDelay  SampleTime=-1
  Unit Delay1 : UnitDelay  SampleTime=-1
  Unit Delay2 : UnitDelay  SampleTime=-1
  Zero-Order Hold : ZeroOrderHold  SampleTime=-1
  Zero-Order Hold1 : ZeroOrderHold  SampleTime=-1
  Zero-Order Hold2 : ZeroOrderHold  SampleTime=-1
  igd_u_pu : Outport
  igd_v_pu : Outport  Port=2
  igd_w_pu : Outport  Port=3
  wires:
  Quantizer1/1 -> Unit Delay1/1
  Quantizer4/1 -> Unit Delay/1
  Quantizer2/1 -> Unit Delay2/1
  ig_u_pu/1 -> Zero-Order Hold/1
  ig_v_pu/1 -> Zero-Order Hold1/1
  ig_w_pu/1 -> Zero-Order Hold2/1
  Unit Delay/1 -> Gain4/1
  Unit Delay1/1 -> Gain5/1
  Unit Delay2/1 -> Gain6/1
  Gain4/1 -> igd_u_pu/1
  Gain5/1 -> igd_v_pu/1
  Gain6/1 -> igd_w_pu/1
  Zero-Order Hold/1 -> Quantizer4/1
  Zero-Order Hold1/1 -> Quantizer1/1
  Zero-Order Hold2/1 -> Quantizer2/1

== system afe_dqctrl_param/afe_dq_mod1/AFE_control/afe_control/acquisitions/is afe quantizzation and one step delay/is afe quantizzation and one step delay ==
  is_u_pu : Inport
  is_v_pu : Inport  Port=2
  is_w_pu : Inport  Port=3
  Quantizer : Quantizer  QuantizationInterval=param.meas.adc_quantization
  Quantizer1 : Quantizer  QuantizationInterval=param.meas.adc_quantization
  Quantizer2 : Quantizer  QuantizationInterval=param.meas.adc_quantization
  Unit Delay : UnitDelay  SampleTime=-1
  Unit Delay1 : UnitDelay  SampleTime=-1
  Unit Delay2 : UnitDelay  SampleTime=-1
  Zero-Order Hold : ZeroOrderHold  SampleTime=-1
  Zero-Order Hold1 : ZeroOrderHold  SampleTime=-1
  Zero-Order Hold2 : ZeroOrderHold  SampleTime=-1
  isd_u_pu : Outport
  isd_v_pu : Outport  Port=2
  isd_w_pu : Outport  Port=3
  wires:
  Unit Delay/1 -> isd_u_pu/1
  Unit Delay1/1 -> isd_v_pu/1
  Unit Delay2/1 -> isd_w_pu/1
  Quantizer/1 -> Unit Delay/1
  Quantizer1/1 -> Unit Delay1/1
  Quantizer2/1 -> Unit Delay2/1
  is_u_pu/1 -> Zero-Order Hold/1
  is_v_pu/1 -> Zero-Order Hold1/1
  is_w_pu/1 -> Zero-Order Hold2/1
  Zero-Order Hold/1 -> Quantizer/1
  Zero-Order Hold1/1 -> Quantizer1/1
  Zero-Order Hold2/1 -> Quantizer2/1

== system afe_dqctrl_param/afe_dq_mod1/AFE_control/afe_control/acquisitions/phase_compensation_1/alignment_eval_afe1 ==
  local_time : Inport
  master_time : Inport  Port=2
  Constant : Constant  Value=0
  Gain : Gain  Gain=-1
  Sum : Sum  Inputs=|+-
  pi : Subsystem  mask{kp=param.ctrl.kp_align, ki=param.ctrl.ki_align*param.glb_time.ts_afe, lim_up=param.ctrl.lim_up_align, lim_down=param.ctrl.lim_down_align}
      mask prompts: ki "ki*ts"
      mask Display:
      | disp('pi()');
      | port_label('input', 1, 'u_ref');
      | port_label('input', 2, 'u');
      | port_label('output', 1, 'y');
  dp : Outport
  wires:
  master_time/1 -> Sum/1
  Sum/1 -> Gain/1
  Constant/1 -> pi/1(u_ref)
  local_time/1 -> Sum/2
  Gain/1 -> pi/2(u)
  pi/1(y) -> dp/1

== system afe_dqctrl_param/afe_dq_mod1/AFE_control/afe_control/acquisitions/ug afe quantizzation and one step delay/ug afe quantizzation and one step delay ==
  ug_u_pu : Inport
  ug_v_pu : Inport  Port=2
  ug_w_pu : Inport  Port=3
  Quantizer1 : Quantizer  QuantizationInterval=param.meas.adc_quantization
  Quantizer2 : Quantizer  QuantizationInterval=param.meas.adc_quantization
  Quantizer4 : Quantizer  QuantizationInterval=param.meas.adc_quantization
  Unit Delay : UnitDelay  SampleTime=-1
  Unit Delay1 : UnitDelay  SampleTime=-1
  Unit Delay2 : UnitDelay  SampleTime=-1
  Zero-Order Hold : ZeroOrderHold  SampleTime=-1
  Zero-Order Hold1 : ZeroOrderHold  SampleTime=-1
  Zero-Order Hold2 : ZeroOrderHold  SampleTime=-1
  ugd_u_pu : Outport
  ugd_v_pu : Outport  Port=2
  ugd_w_pu : Outport  Port=3
  wires:
  Unit Delay/1 -> ugd_u_pu/1
  Unit Delay1/1 -> ugd_v_pu/1
  Unit Delay2/1 -> ugd_w_pu/1
  Quantizer4/1 -> Unit Delay/1
  Quantizer1/1 -> Unit Delay1/1
  Quantizer2/1 -> Unit Delay2/1
  ug_w_pu/1 -> Zero-Order Hold2/1
  ug_v_pu/1 -> Zero-Order Hold1/1
  ug_u_pu/1 -> Zero-Order Hold/1
  Zero-Order Hold/1 -> Quantizer4/1
  Zero-Order Hold1/1 -> Quantizer1/1
  Zero-Order Hold2/1 -> Quantizer2/1

== system afe_dqctrl_param/afe_dq_mod1/AFE_control/afe_control/current_ctrl/dq_vector_pi/bounder1 ==
  md : Inport
  m_1 : Inport  Port=2
  m : Inport  Port=3
  Constant : Constant
  Constant1 : Constant  Value=0
  Divide : Product
  Switch : Switch  Threshold=1  SaturateOnIntegerOverflow=off  InputSameDT=off
  Switch1 : Switch  Threshold=1  SaturateOnIntegerOverflow=off  InputSameDT=off
  md_sat : Outport  VectorParamsAs1DForOutWhenUnconnected=off
  clip : Outport  Port=2  VectorParamsAs1DForOutWhenUnconnected=off
  wires:
  md/1 -> Switch1/3, Divide/2
  m_1/1 -> Divide/1
  Divide/1 -> Switch1/1
  Switch1/1 -> md_sat/1
  Switch/1 -> clip/1
  m/1 -> Switch/2, Switch1/2
  Constant/1 -> Switch/1
  Constant1/1 -> Switch/3

== system afe_dqctrl_param/afe_dq_mod1/AFE_control/afe_control/current_ctrl/dq_vector_pi/bounder2 ==
  m : Inport
  m_1 : Inport  Port=2
  mq : Inport  Port=3
  Constant : Constant
  Constant1 : Constant  Value=0
  Divide : Product
  Switch : Switch  Threshold=1  SaturateOnIntegerOverflow=off  InputSameDT=off
  Switch1 : Switch  Threshold=1  SaturateOnIntegerOverflow=off  InputSameDT=off
  mq_sat : Outport  VectorParamsAs1DForOutWhenUnconnected=off
  clip : Outport  Port=2  VectorParamsAs1DForOutWhenUnconnected=off
  wires:
  Constant1/1 -> Switch/3
  Constant/1 -> Switch/1
  m/1 -> Switch1/2, Switch/2
  Switch/1 -> clip/1
  Switch1/1 -> mq_sat/1
  Divide/1 -> Switch1/1
  m_1/1 -> Divide/1
  mq/1 -> Divide/2, Switch1/3

== system afe_dqctrl_param/afe_dq_mod1/AFE_control/afe_control/current_ctrl/dq_vector_pi/pi_d ==
  id_tilde : Inport
  clip : Inport  Port=2
  1/Ti : Gain  Gain=param.afe.dq_vector_pi.kp_i  SaturateOnIntegerOverflow=on  OutDataTypeStr=Inherit: Same as input  ParamDataTypeStr=Inherit: Same as input
  Constant : Constant  Value=0
  Sum2 : Sum  Inputs=+-  SaturateOnIntegerOverflow=on
  Sum4 : Sum  SaturateOnIntegerOverflow=on
  Sum5 : Sum  SaturateOnIntegerOverflow=on
  Switch1 : Switch  Threshold=0.5  SaturateOnIntegerOverflow=off  InputSameDT=off
  Switch2 : Switch  Threshold=0.5  SaturateOnIntegerOverflow=off  InputSameDT=off
  Unit Delay1 : UnitDelay  SampleTime=-1
  Unit Delay2 : UnitDelay  SampleTime=-1
  kp1 : Gain  Gain=param.ctrl.CTRPIFF_CLIP_RELEASE*param.glb_time.ts_inv  SaturateOnIntegerOverflow=on  OutDataTypeStr=Inherit: Same as input  ParamDataTypeStr=Inherit: Same as input
  kp2 : Gain  Gain=param.afe.dq_vector_pi.ki_i*param.glb_time.ts_inv  SaturateOnIntegerOverflow=on  OutDataTypeStr=Inherit: Same as input  ParamDataTypeStr=Inherit: Same as input
  ud_out : Outport  VectorParamsAs1DForOutWhenUnconnected=off
  wires:
  id_tilde/1 -> kp2/1, 1/Ti/1
  Sum5/1 -> ud_out/1
  Switch1/1 -> Unit Delay2/1
  Sum4/1 -> Sum5/2, Switch1/3
  kp1/1 -> Sum2/2
  Sum2/1 -> Switch1/1
  Unit Delay2/1 -> Sum4/2, kp1/1, Sum2/1
  1/Ti/1 -> Sum5/1
  Switch2/1 -> Sum4/1
  kp2/1 -> Switch2/3
  clip/1 -> Unit Delay1/1
  [clip] -> Switch2/2
  [clip] -> Switch1/2
  Constant/1 -> Switch2/1
  Unit Delay1/1 -> [clip]

== system afe_dqctrl_param/afe_dq_mod1/AFE_control/afe_control/current_ctrl/dq_vector_pi/pi_q ==
  iq_tilde : Inport
  clip : Inport  Port=2
  1/Ti : Gain  Gain=param.afe.dq_vector_pi.kp_i  SaturateOnIntegerOverflow=on  OutDataTypeStr=Inherit: Same as input  ParamDataTypeStr=Inherit: Same as input
  Constant : Constant  Value=0
  Sum2 : Sum  Inputs=+-  SaturateOnIntegerOverflow=on
  Sum4 : Sum  SaturateOnIntegerOverflow=on
  Sum5 : Sum  SaturateOnIntegerOverflow=on
  Switch1 : Switch  Threshold=0.5  SaturateOnIntegerOverflow=off  InputSameDT=off
  Switch2 : Switch  Threshold=0.5  SaturateOnIntegerOverflow=off  InputSameDT=off
  Unit Delay1 : UnitDelay  SampleTime=-1
  Unit Delay2 : UnitDelay  SampleTime=-1
  kp1 : Gain  Gain=param.ctrl.CTRPIFF_CLIP_RELEASE*param.glb_time.ts_inv  SaturateOnIntegerOverflow=on  OutDataTypeStr=Inherit: Same as input  ParamDataTypeStr=Inherit: Same as input
  kp2 : Gain  Gain=param.afe.dq_vector_pi.ki_i*param.glb_time.ts_inv  SaturateOnIntegerOverflow=on  OutDataTypeStr=Inherit: Same as input  ParamDataTypeStr=Inherit: Same as input
  Vqs_out : Outport  VectorParamsAs1DForOutWhenUnconnected=off
  wires:
  Constant/1 -> Switch2/1
  [clip] -> Switch1/2
  [clip] -> Switch2/2
  clip/1 -> Unit Delay1/1
  kp2/1 -> Switch2/3
  Switch2/1 -> Sum4/1
  1/Ti/1 -> Sum5/1
  Unit Delay2/1 -> Sum2/1, kp1/1, Sum4/2
  Sum2/1 -> Switch1/1
  kp1/1 -> Sum2/2
  Sum4/1 -> Sum5/2, Switch1/3
  Switch1/1 -> Unit Delay2/1
  iq_tilde/1 -> 1/Ti/1, kp2/1
  Unit Delay1/1 -> [clip]
  Sum5/1 -> Vqs_out/1

== system afe_dqctrl_param/afe_dq_mod1/AFE_control/afe_control/current_ctrl/dq_vector_pi/switch ==
  clip 1 : Inport
  clip 2 : Inport  Port=2
  Constant4 : Constant
  Constant5 : Constant  Value=0
  Sum1 : Sum  SaturateOnIntegerOverflow=on
  Switch : Switch  Threshold=0.5  SaturateOnIntegerOverflow=off  InputSameDT=off
  clip : Outport  VectorParamsAs1DForOutWhenUnconnected=off
  wires:
  Constant5/1 -> Switch/3
  Switch/1 -> clip/1
  Constant4/1 -> Switch/1
  Sum1/1 -> Switch/2
  clip 1/1 -> Sum1/1
  clip 2/1 -> Sum1/2

== system afe_dqctrl_param/afe_dq_mod1/AFE_control/afe_control/current_ctrl/dq_vector_pi/vector lenght ==
  md : Inport
  mq : Inport  Port=2
  Math Function : Math  Operator=magnitude^2  SignedPower=on
  Math Function1 : Math  Operator=magnitude^2  SignedPower=on
  Math Function2 : Math  Operator=reciprocal  SignedPower=on
  Sqrt : Sqrt
  Sum5 : Sum  SaturateOnIntegerOverflow=on
  m_1 : Outport  VectorParamsAs1DForOutWhenUnconnected=off
  m : Outport  Port=2  VectorParamsAs1DForOutWhenUnconnected=off
  wires:
  Sqrt/1 -> m/1, Math Function2/1
  mq/1 -> Math Function1/1
  Math Function1/1 -> Sum5/2
  Math Function/1 -> Sum5/1
  Sum5/1 -> Sqrt/1
  Math Function2/1 -> m_1/1
  md/1 -> Math Function/1

== system afe_dqctrl_param/afe_dq_mod1/AFE_control/afe_control/current_ctrl/zero_current_ctrl/iz ==
  Demux : Demux  Outputs=3
  Gain : Gain  Gain=1/3
  Sum : Sum  Inputs=+++
  iz : Outport
  wires:
  Sum/1 -> Gain/1
  Demux/1 -> Sum/1  "is_a"
  [isd_abc_pu] -> Demux/1
  Demux/3 -> Sum/3  "is_c"
  Demux/2 -> Sum/2  "is_b"
  Gain/1 -> iz/1

== system afe_dqctrl_param/afe_dq_mod1/AFE_control/afe_control/current_ctrl/zero_current_ctrl/zero_sequence_current_ctrl ==
  iz : Inport
  1/Ti : Gain  Gain=param.afe.ctrl.kp_is_z  SaturateOnIntegerOverflow=on  OutDataTypeStr=Inherit: Same as input  ParamDataTypeStr=Inherit: Same as input
  Constant1 : Constant  Value=0
  Gain : Gain
  Saturation : Saturate  UpperLimit=1  LowerLimit=-1
  Sum1 : Sum  Inputs=+++  SaturateOnIntegerOverflow=on
  Sum2 : Sum  Inputs=-+  SaturateOnIntegerOverflow=on
  Sum3 : Sum  Inputs=-+  SaturateOnIntegerOverflow=on
  Unit Delay4 : UnitDelay  SampleTime=-1
  iz_tracking : Scope  NumInputPorts=3
      settings: ActiveDisplayYMinimum=-1  ActiveDisplayYMaximum=1  DataLoggingVariableName=ScopeData8
  kp : Gain  Gain=param.afe.ctrl.ki_is_z*param.glb_time.ts_afe  SaturateOnIntegerOverflow=on  OutDataTypeStr=Inherit: Same as input  ParamDataTypeStr=Inherit: Same as input
  ugamma_afe : Outport
  tag scope: iz_ctrl_out=scoped, iz_pu=scoped, iz_pu_ref=scoped
  wires:
  1/Ti/1 -> Sum1/1, Sum3/1
  kp/1 -> Sum1/2
  Sum3/1 -> Unit Delay4/1
  Unit Delay4/1 -> Sum1/3
  Constant1/1 -> [iz_pu_ref], iz_tracking/1, Sum2/2  "iz_pu_ref"
  iz/1 -> [iz_pu], iz_tracking/2, Sum2/1  "iz_pu"
  Sum2/1 -> kp/1, 1/Ti/1
  Sum1/1 -> Saturation/1
  Saturation/1 -> Gain/1, [iz_ctrl_out], iz_tracking/3, Sum3/2  "iz_ctrl_out"
  Gain/1 -> ugamma_afe/1

== system afe_dqctrl_param/afe_dq_mod1/AFE_control/afe_control/grid_voltage_phase_lock_loops/FHT-PLL/pll_stageA ==
  gamma_grid : Inport
  ug_abc_pu : Inport  Port=2
  Demux : Demux  Outputs=3
  Math Function : Math  Operator=magnitude^2  SignedPower=on
  Math Function1 : Math  Operator=magnitude^2  SignedPower=on
  Reciprocal Sqrt : Sqrt  Operator=rSqrt
  Saturation : Saturate  UpperLimit=inf  LowerLimit=0.02
  Sum : Sum  Inputs=|++
  filter_and_transformation : Subsystem
  sequences : Subsystem
  u_grid_xi : Outport  VectorParamsAs1DForOutWhenUnconnected=off
  u_grid_eta : Outport  Port=2  VectorParamsAs1DForOutWhenUnconnected=off
  tag scope: Vgrid_unorm_fht=scoped
  wires:
  gamma_grid/1 -> sequences/3(phase_angle)
  sequences/2(u_grid_eta) -> u_grid_eta/1
  sequences/1(u_grid_xi) -> u_grid_xi/1
  ug_abc_pu/1 -> Demux/1
  Demux/1 -> filter_and_transformation/1(ug_a)
  Demux/2 -> filter_and_transformation/2(ug_b)
  Demux/3 -> filter_and_transformation/3(ug_c)
  filter_and_transformation/1(ug_alpha) -> Math Function/1, sequences/1(u_grid_alpha)
  filter_and_transformation/2(ug_beta) -> Math Function1/1, sequences/2(u_grid_beta)
  Math Function/1 -> Sum/1
  Math Function1/1 -> Sum/2
  Sum/1 -> Saturation/1
  Reciprocal Sqrt/1 -> [Vgrid_unorm_fht]
  Saturation/1 -> Reciprocal Sqrt/1
